simulink model "EMT"  (R2024b)
settings: Solver=ode5  StartTime=0.0  StopTime=1500  FixedStep=0.002  RelTol=1e-3
PreLoadFcn:
  | parameter;
InitFcn:
  | parameter;
StopFcn:
  | save('result.mat');
values from neighbouring files (symbols this model uses):
  A = 7.3    [parameter.m]
  a11 = (1+k1)*(1+k2)/k1/k2/iq    (= 1.54241568346)    [parameter.m]
  a11_L = a11    (= 1.54241568346)    [parameter.m]
  a12 = -(1+k1+k2)*(1+k3)/k1/k2    (= -3.86074191629)    [parameter.m]
  a12_L = a11*(1+k3+k4)/(1+k3)    (= 2.43173643789)    [parameter.m]
  a21 = -(1+k2)/k1/iq    (= -1.04963112005)    [parameter.m]
  a22 = (1+k1+k2)/k1    (= 2.46948356808)    [parameter.m]
  B = 2.71    [parameter.m]
  b11 = 0    [parameter.m]
  b12 = (1+k3)    (= 3.33)    [parameter.m]
  b21 = (1+k2)/iq    (= 2.23571428571)    [parameter.m]
  b22 = -k2    (= -2.13)    [parameter.m]
  C1_shift = 200    [parameter.m]
  Cb = 70    [parameter.m]
  Cd = 0.6    [parameter.m]
  eff_generator = eff_motor    [parameter.m]
  eff_motor = [0.80 0.80 0.84 0.84 0.83 0.85 0.83 0.83 0.83 0.80 0.80 0.80 ... (first row only)    [parameter.m]
  ele_map = [10.00,11.46,14.13,19.24,20.94,23.21,20.29,20.23,22.28,17.66,16.24,18.95,20.79,16.98,18.22,16.52,18.29,20.67,20.82,23.14,23.36,21.30,17.71,20.26,19.53,21.18,23.13,22.79,19.35,16.77,20.50,19.02,20.56,21.90,23.91,20.40,18.45,22.70,22.38,22.48,21.84,17.76,20.13,22.61,19.35,19.36,21.56,20.37,18.38,17.96,18.38,17.24,18.99,22.31,23.50,18.24,22.11,20.73,20.35,18.91,22.88,20.92,18.75,16.85,21.94,17.80,19. ...(+2007 chars)    [parameter.m]
  Fb_max = 5.5*mass    (= 247500)    [parameter.m]
  ic = 4.42    [parameter.m]
  JA = 0.4    [parameter.m]
  JB = JA    (= 0.4)    [parameter.m]
  Jc3r4 = 1e-2    (= 0.01)    [parameter.m]
  Je = 2.5    [parameter.m]
  Jh = 1e-2    (= 0.01)    [parameter.m]
  kh = 2.88    [parameter.m]
  kt = 1.83    [parameter.m]
  L = 4.472    [parameter.m]
  mass = 45000    [parameter.m]
  miu_max = 0.8    [parameter.m]
  n_generator = n_motor    [parameter.m]
  n_motor = [0 0.1 0.25 0.4 0.55 0.7 0.85 1 1.15 1.3 1.45 2.2]*3185    [parameter.m]
  nA_map = [-6000:50:-3250 -3200 0 3200 3250:50:6000]    [parameter.m]    (also in plot_result.m = [-7000:50:-3250 -3200 0 3200 3250:50:7000])
  nA_max = max(nA_map)    [parameter.m]
  nA_min = min(nA_map)    [parameter.m]
  nB_map = nA_map    [parameter.m]    (also in plot_result.m = [-7000:50:-3250 -3200 0 3200 3250:50:7000])
  nB_max = nA_max    [parameter.m]
  nB_min = nA_min    [parameter.m]
  ne_idl = 3000    [parameter.m]
  ne_map = [1600,1700,1800,1900,2000,2100,2200,2300,2400,2500,2600,2700,2800,2900,3000,3100,3200,3300,3400,3500,3600,3700,3800,3900,4000,4100,4200,4500]    [parameter.m]
  ne_max = 4200    [parameter.m]
  ne_min = 1600    [parameter.m]
  ne_start = 200    [parameter.m]
  nZ_map = [-8000:50:-4850 -4800 0 4800 4850:50:8000]    [parameter.m]
  Pb_epr = [-45 -45 -40 -30 0 30 40 45 45]    [parameter.m]
  Pb_max = [0 40 45 45 45]    [parameter.m]
  Pb_min = [-45 -45 -45 -40 0]    [parameter.m]
  Pe_ass = 210+20    (= 230)    [parameter.m]
  Pe_max = 1103    [parameter.m]
  PN0 = 0    [parameter.m]
  R_map = [0.90 0.89 0.90 0.91 0.92 0.93 0.94 0.95 0.96 0.97 0.98]/10    [parameter.m]
  rz = 0.318    [parameter.m]
  SOC0 = 60    [parameter.m]
  SOC_epr = [30 31 50 59 60 61 70 79 80]    [parameter.m]
  SOC_map = 0:10:100    [parameter.m]
  T_generator = T_motor    [parameter.m]
  T_motor = [0 0.3 0.8 1.3 1.8 2.3 2.8]/1.8*1110    [parameter.m]
  TA_max_map = [370*9549./(6000:-50:3250) 1110 1110 1110 370*9549./(3250:50:6000)]    [parameter.m]    (also in plot_result.m = [370*9549./(7000:-50:3250) 1100 1100 1100 370*9549./(3250:50)
  TA_min_map = -TA_max_map    [parameter.m]
  TAf = 0    [parameter.m]
  TB_max_map = TA_max_map    [parameter.m]    (also in plot_result.m = [370*9549./(7000:-50:3250) 1110 1110 1110 370*9549./(3250:50)
  TB_min_map = TA_min_map    [parameter.m]
  TBf = TAf    (= 0)    [parameter.m]
  Te_map = [0,599,798,998,1168,1324,1495,1660,1822,1970,2106,2235,2355,2458,2508,2543,2565,2606,2613,2649,2658,2689,2701,2707,2719,2724,2728,2740,2743,2754]    [parameter.m]
  Te_max_map = [1168,1324,1495,1660,1822,1970,2106,2235,2355,2458,2543,2606,2658,2701,2728,2743,2754,2743,2740,2724,2719,2707,2689,2649,2613,2565,2508,998]    [parameter.m]
  Te_start = 1600    [parameter.m]
  Tef = 100    [parameter.m]
  Time = 0:0.1:200    [parameter.m]
  Time_ele = 0:4:1600    [parameter.m]
  TS_A = 0.2    [parameter.m]
  TS_B = TS_A    (= 0.2)    [parameter.m]
  TS_C0 = 0.2    [parameter.m]
  TS_C1 = 0.2    [parameter.m]
  Ts_e = 0.1    [parameter.m]
  TS_Z1 = 0.2    [parameter.m]
  TS_Z2 = 0.2    [parameter.m]
  TZ_max_map = [450*9549./(8000:-50:4850) 1000 1000 1000 450*9549./(4850:50:8000)]    [parameter.m]
  TZ_min_map = -TZ_max_map    [parameter.m]
  Uoc_map = [3.258,3.668,3.733,3.783,3.833,3.877,3.912,3.941,3.973,4.013,4.200]*250    [parameter.m]
  v_cyc = 0.*(0<=Time&Time<11)+(3.75.*Time-41.25).*(11<=Time&Time<15)+15.*(15<=Time&Time<23)+(-3.*Time+84).*(23<=Time&Time<28)+0.*(28<=Time&Time<49)+(8.*Time/3-392/3).*(49<=Time&Time<61)+32.*(61<=Time&Time<85)+(-32.*Time/11+3072/11).*(85<=Time&Time<96)+0.*(96<=Time&Time<117)+(25.*Time/13-2925/13).*(117<=Time&Time<143)+50.*(143<=Time&Time<155)+(-15.*Time/8+2725/8).*(155<=Time&Time<163)+35.*(163<=Time&Time<17 ...(+70 chars)    [parameter.m]
  V_Shift12 = 32    [parameter.m]
  V_Shift21 = 25    [parameter.m]
  Voltage_epr = [750 760 900 1000 1050]    [parameter.m]
  Y_engine = 0.955    [parameter.m]
  Yc = 0.98    [parameter.m]
  Yh = 0.96    [parameter.m]
  Z1_shift = 200    [parameter.m]
  Z2_shift = 200    [parameter.m]
undefined symbols (not defined in the file or in its folder): sigbuilder_block
libraries: fl_lib x82, nesl_utility x55, simulink x49, sdl_lib x10, simulink_need_slupdate x6, powerlib_extras x1
(part 6 of 6)

== matlab function EMT/Control Unit/Control/Power Distribution/Optimal Power Distribution/Optimization  ==
  data: u input; y output
function y = fcn(u)
%#codegen
Pe_com=u(1);pedal=u(2);ZD=u(3);stage=u(4);ne_act=u(5);ne_max=u(6);ne_min=u(7);
no_act=u(8);Te_max=u(9);Te_min=u(10);TA_max=u(11);TA_min=u(12);TB_max=u(13);
TB_min=u(14);PN_com=u(15);PN_max=u(16);PN_min=u(17);PZ_com=u(18);sd_ne=u(19);
%转速转矩关系
a11=1.5424;a12=-3.8607;%EVT1模式下nA表达式的系数nA=a11*ne+a12*no
a11_L=1.5424;a12_L=2.4317;%EVT1_L模式下nA表达式的系数nA=a11_L*ne+a12_L*no
b11=0;b12=3.3300;%EVT1模式下nB表达式的系数nB=b11*ne+b12*no
b11_L=0;b12_L=7.8036;%EVT1模式下nB表达式的系数nB=b11*ne+b12*no
a21=-1.0496;a22=2.4695;%EVT2模式下nA表达式的系数nA=a21*ne+a22*no
b21=2.2357;b22=-2.1300;%EVT2模式下nB表达式的系数nB=b21*ne+b22*no
e11=-1.5424;e12=0;%EVT1模式下Te表达式的系数Te=e11*TA+e12*TB
f11=-3.8607;f12=3.3300;%EVT1模式下To表达式的系数To=f11*TA+f12*TB
e21=1.0496;e22=-2.2357;%EVT2模式下Te表达式的系数Te=e21*TA+e22*TB
f21=2.4695;f22=-2.1300;%EVT2模式下To表达式的系数To=f21*TA+f22*TB
kq=2.17;YE=0.75;YA=0.8;YB=0.8;%平均效率
if pedal>0.99&&no_act<49.67*50
    TA_max=1.5*TA_max;TA_min=1.5*TA_min;
    TB_max=1.5*TB_max;TB_min=1.5*TB_min;
else
end
if stage<3
    nA=a11*ne_act+a12*no_act;
    nB=b11*ne_act+b12*no_act;
elseif stage<4
    nA=a21*ne_act+a22*no_act;
    nB=b21*ne_act+b22*no_act;
else
    nA=a11_L*ne_act+a12_L*no_act;
    nB=b11_L*ne_act+b12_L*no_act;
end
%发动机燃油经济性曲线
Peg=[0,100,120,140,160,180,200,220,240,260,280,300,320,340,360,380,400,420,440,460,480,500,520,540,560,580,600,620,640,660,680,700,720,740,760,780,800,820,840,860,880,900,920,940,960,980,1000,1020,1040,1060,1080,1100,1200];
neg=[1600,1600,1800,1860,1910,2000,2001,2200,2300,2301,2400,2450,2610,2611,2612,2613,2700,2701,2702,2730,2790,2880,2900,2901,2902,2903,3200,3201,3202,3203,3204,3205,3206,3207,3300,3301,3302,3310,3350,3390,3420,3500,3501,3700,3701,3702,3760,3761,3810,4180,4200,4200,4200];
Pe_com=min(Pe_com,max(Peg));
Pe_com=max(Pe_com,min(Peg));
ne_ref=interp1(Peg,neg,Pe_com);
ne_idl=3000;%发动机启动转速
V_Shift12=32;%EVT1到EVT2的换段车速(km/h)
V_Shift21=25;%EVT2到EVT1的换段车速(km/h)
alpha=max(pedal,0);
V_Shift12=V_Shift12-5*(1-alpha);
V_Shift21=V_Shift21+5*alpha;
if stage<3&&no_act>49.67*(V_Shift12-2)
    ne_ref=max(2.442*no_act,ne_ref);
elseif stage>1&&no_act<49.67*(V_Shift21+2)
    ne_ref=min(2.442*no_act,ne_ref);
elseif pedal<0
    ne_ref=2.442*no_act;   
else
end
if pedal>0.8&&ne_max<4200&&no_act<49.67*10
    ne_max=ne_max-500;
else
end
ne_min=max(ne_idl,ne_min);ne_max=min(4200,ne_max);
ne_min=max(ne_act-100,ne_min);ne_max=min(ne_act+500,ne_max);
ne_ref=max(ne_ref,ne_min);ne_ref=min(ne_ref,ne_max);
ne_ref0=ne_ref;
if pedal>0
    ne_ref=ne_ref+sd_ne;
else
end
% x_ne=[-500 -200 -100 -50 0 50 100 200 500];
% x_Te=[0.1 0.2 0.5 0.8 1 1.5 2.0 5.0 10];
x_ne=[-200 0 200];
x_Te=[0.6 1 2.0];
dne=ne_ref-ne_act;dne=min(dne,200);dne=max(dne,-200);
x_ne=interp1(x_ne,x_Te,dne);
if ne_act==0
    Te_ref=Te_max;
else
    Te_ref=9549*Pe_com/ne_act;
end
Te_ref=max(Te_ref,200);
Te_ref=x_ne*Te_ref;
Te_ref=max(Te_ref,Te_min);Te_ref=min(Te_ref,Te_max);
Te1=linspace(Te_ref,Te_min,10);Te2=linspace(Te_ref,Te_max,10);
Te=[Te1 Te2];L_Te=length(Te);
TA=linspace(TA_min,TA_max,20);L_TA=length(TA);
TB=linspace(TB_min,TB_max,20);L_TB=length(TB);
TA0=zeros(1,L_TA*L_TB);TB0=zeros(1,L_TA*L_TB);
for i=1:L_TA
    for j=1:L_TB
        TA0((j-1)*L_TA+i)=TA(i);
        TB0((j-1)*L_TA+i)=TB(j);
    end
end
TA=TA0;TB=TB0;
if ZD==1
    if stage==3
        Tef=(e21.*TA+e22.*TB);
        To=(f21.*TA+f22.*TB);
    else
        Tef=(e11.*TA+e12.*TB);
        To=(f11.*TA+f12.*TB);
    end
else
    if stage==3
        Tef=(e21.*TA+e22.*TB)/kq;
        To=(f21.*TA+f22.*TB)/kq;
    else
        Tef=(e11.*TA+e12.*TB)/kq;
        To=(f11.*TA+f12.*TB)/kq;
    end
end
Tef=Tef*YE;
PA=TA*nA/9549;PB=TB*nB/9549;
PN=PA.*YA.^sign(-PA)+PB.*YB.^sign(-PB);
PN_com=PN_com-PZ_com;
TA_ref=0;TB_ref=0;
J0=1e10;NN_Te=0;
NN_ne=zeros(L_Te,L_TA*L_TB);
NN_PN0=zeros(L_Te,L_TA*L_TB);
NN_PN1=zeros(L_Te,L_TA*L_TB);
for i=1:L_Te    
    for j=1:L_TA*L_TB
        if (PN(j)<3*PN_min&&PN(j)-PN_com<3*PN_min)||(PN(j)>3*PN_max&&PN(j)-PN_com>3*PN_max)
            continue;
        else
        end
        NN_PN0(i,j)=1;         
        if dne>10
            if Tef(j)*x_ne>Te(i)
                continue;
            else
            end     
        elseif dne<-10
            if Tef(j)*x_ne<Te(i)
                continue;
            else
            end
        else
        end
        NN_ne(i,j)=1;
        if PN(j)-PN_com<3*PN_min||PN(j)-PN_com>3*PN_max
            continue;
        else
        end
        NN_PN1(i,j)=1;
        if PN(j)-PN_com<PN_min||PN(j)-PN_com>PN_max
            continue;
        else
        end
        if PN_com>0
            if PN(j)<0
                continue;
            else
            end
        elseif PN_com<0 
            if PN(j)>0
                continue;
            else
            end
        else
        end
        if pedal>=0.9
            J1=0;
        elseif pedal<=0
            J1=PN(i);
        else
            J1=abs(PN(j)-PN_com);
        end
        if pedal<=0
            J2=0;
        else
            J2=-To(j)*ne_ref/9549;
        end
        J=J1+J2;
        if J<J0
            J0=J;
            Te_ref=Te(i);TA_ref=TA(j);TB_ref=TB(j);
            NN_Te=1;
        else
        end
    end
    if NN_Te==1
        break;
    else
    end
    for j=1:L_TA*L_TB
        if NN_PN1(i,j)==0
            continue;
        else
        end
        if pedal>=0.9
            J1=0;
        elseif pedal<=0
            J1=PN(i);
        else
            J1=abs(PN(j)-PN_com);
        end
        if pedal<=0
            J2=0;
        else
            J2=-To(j)*ne_ref/9549;
        end
        J=J1+J2;
        if J<J0
            J0=J;
            Te_ref=Te(i);TA_ref=TA(j);TB_ref=TB(j);
            NN_Te=1;
        else
        end
    end
    if NN_Te==1
        break;
    else
    end
end
if NN_Te==0
    for i=1:L_Te    
        for j=1:L_TA*L_TB
            if NN_ne(i,j)==0
                continue;
            else
            end
            if PN_com<0
                if PN(j)-PN_com>3*PN_max
                    continue;
                else
                end
                J1=PN(j);
            else
                if PN(j)-PN_com<3*PN_min
                    continue;
                else
                end
                J1=-PN(j);
            end
            if pedal<=0
                J2=0;
            else
                J2=-To(j)*ne_ref/9549;
            end
            J=100*J1+J2;
            if J<J0
                J0=J;
                Te_ref=Te(i);TA_ref=TA(j);TB_ref=TB(j);

            else
            end 
        end
    end
else
end
if NN_Te==0
    if ne_ref>ne_act
        Te_ref=Te_max;
    else
        Te_ref=Te_min;
    end
    for j=1:L_TA*L_TB
        if  NN_PN0(i,j)==0
            continue;
        else
        end
        if ne_ref>ne_act
            J1=Tef(j);
        else
            J1=-Tef(j);
        end
        if pedal<=0
            J2=0;
        else
            J2=-To(j);
        end
        J=100*J1+J2;
        if J<J0
            J0=J;
            Te_ref=Te(i);TA_ref=TA(j);TB_ref=TB(j);
            NN_Te=1;
        else
        end 
    end
else
end
if NN_Te==0
    for i=1:L_Te    
        for j=1:L_TA*L_TB
            if dne>10
                if Tef(j)*x_ne>Te(i)
                    continue;
                else
                end     
            elseif dne<-10
                if Tef(j)*x_ne<Te(i)
                    continue;
                else
                end
            else
            end
            if PN(j)<PN_min
                J1=-PN(j);
            elseif PN(j)>PN_max
                J1=PN(j);
            else
                J1=abs(PN(j)-PN_com);
            end            
            if pedal<=0
                J2=0;
            else
                J2=-To(j)*ne_ref/9549;
            end
            if ne_ref>ne_act
                J3=Tef(j)*ne_ref/9549;
            else
                J3=-Tef(j)*ne_ref/9549;
            end
            J=J1+J2+100*J3;
            if J<J0
                J0=J;
                Te_ref=Te(i);TA_ref=TA(j);TB_ref=TB(j);
                NN_Te=1;
            else
            end 
        end
    end
else
end
if NN_Te==0
    if ne_ref>ne_act
        Te_ref=Te_max;
    else
        Te_ref=Te_min;
    end
    for j=1:L_TA*L_TB
        if PN(j)<3*PN_min&&PN(j)-PN_com<3*PN_min
            J1=-PN(j);
        elseif PN(j)>3*PN_max&&PN(j)-PN_com>3*PN_max
            J1=PN(j);
        else
            J1=abs(PN(j)-PN_com);
        end            
        if pedal<=0
            J2=0;
        else
            J2=-To(j)*ne_ref/9549;
        end
        J=100*J1+J2;
        if J<J0
            J0=J;
            Te_ref=Te(i);TA_ref=TA(j);TB_ref=TB(j);
        else
        end 
    end
else
end
ne_ref=ne_ref0;
y=[ne_ref Te_ref TA_ref TB_ref];
